simulink model "OpenLoopSys"  (Simulink 8.4)
settings: Solver=ode45  StartTime=0.0  StopTime=60.0  RelTol=1e-3
values from neighbouring files (symbols this model uses):
  g = 9.81    [heli.m]
  Je = 2*m1*(l1^2)+m2*(l3^2)    (= 0.0023885)    [heli.m]
  Jt = Je    (= 0.0023885)    [heli.m]
  l1 = 0.110    (= 0.11)    [heli.m]
  l3 = 0.108    [heli.m]
  m1 = 0.0505    [heli.m]
  m2 = 0.100    (= 0.1)    [heli.m]
settings Model: Creator=bjones  LastModifiedBy=bjones
settings DebuggingCC: SolverPrmCheckMsg=none

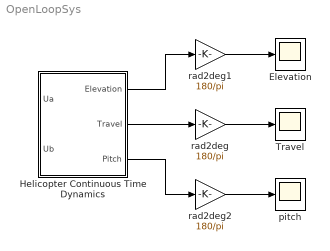
== system OpenLoopSys ==
  Elevation : Scope
      settings: TimeRange=60  YMin=-50  YMax=30  SaveName=elev
  Helicopter Continuous Time Dynamics : Subsystem
  Travel : Scope
      settings: TimeRange=60  YMin=-150  YMax=300  SaveName=trav
  pitch : Scope
      settings: TimeRange=60  YMin=-25  YMax=20  SaveName=pitch
  rad2deg : Gain  Gain=180/pi  SaturateOnIntegerOverflow=on  OutDataTypeStr=Inherit: Same as input  ParamDataTypeStr=Inherit: Same as input
  rad2deg1 : Gain  Gain=180/pi  SaturateOnIntegerOverflow=on  OutDataTypeStr=Inherit: Same as input  ParamDataTypeStr=Inherit: Same as input
  rad2deg2 : Gain  Gain=180/pi  SaturateOnIntegerOverflow=on  OutDataTypeStr=Inherit: Same as input  ParamDataTypeStr=Inherit: Same as input
  wires:
  rad2deg/1 -> Travel/1
  rad2deg1/1 -> Elevation/1
  Helicopter Continuous Time Dynamics/2(Travel) -> rad2deg/1
  Helicopter Continuous Time Dynamics/1(Elevation) -> rad2deg1/1
  rad2deg2/1 -> pitch/1
  Helicopter Continuous Time Dynamics/3(Pitch) -> rad2deg2/1

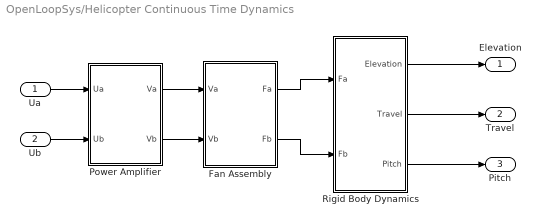
== system OpenLoopSys/Helicopter Continuous Time Dynamics ==
  Ua : Inport
  Ub : Inport  Port=2
  Fan Assembly : Subsystem
  Power Amplifier : Subsystem
  Rigid Body Dynamics : Subsystem
  Elevation : Outport
  Travel : Outport  Port=2
  Pitch : Outport  Port=3
  wires:
  Power Amplifier/1(Va) -> Fan Assembly/1(Va)
  Power Amplifier/2(Vb) -> Fan Assembly/2(Vb)
  Rigid Body Dynamics/1(Elevation) -> Elevation/1
  Rigid Body Dynamics/3(Pitch) -> Pitch/1
  Fan Assembly/2(Fb) -> Rigid Body Dynamics/2(Fb)
  Ua/1 -> Power Amplifier/1(Ua)
  Ub/1 -> Power Amplifier/2(Ub)
  Rigid Body Dynamics/2(Travel) -> Travel/1
  Fan Assembly/1(Fa) -> Rigid Body Dynamics/1(Fa)

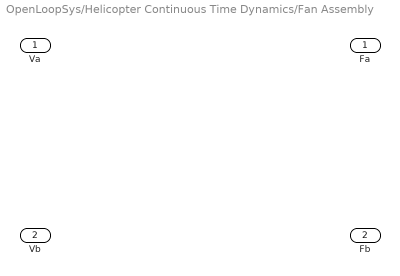
== system OpenLoopSys/Helicopter Continuous Time Dynamics/Fan Assembly ==
  Va : Inport
  Vb : Inport  Port=2
  Fa : Outport
  Fb : Outport  Port=2

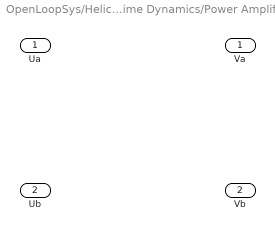
== system OpenLoopSys/Helicopter Continuous Time Dynamics/Power Amplifier ==
  Ua : Inport
  Ub : Inport  Port=2
  Va : Outport
  Vb : Outport  Port=2

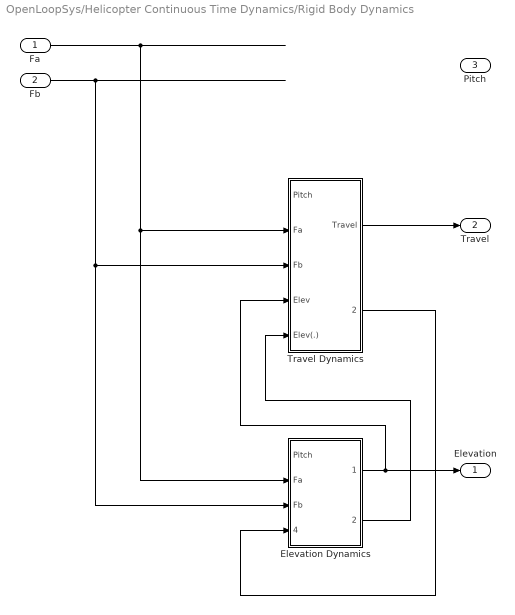
== system OpenLoopSys/Helicopter Continuous Time Dynamics/Rigid Body Dynamics ==
  Fa : Inport
  Fb : Inport  Port=2
  Elevation Dynamics : Subsystem
  Travel Dynamics : Subsystem
  Elevation : Outport
  Travel : Outport  Port=2
  Pitch : Outport  Port=3
  wires:
  Fa/1 -> Travel Dynamics/2(Fa), Elevation Dynamics/2(Fa)
  Fb/1 -> Elevation Dynamics/3(Fb), Travel Dynamics/3(Fb)
  Travel Dynamics/1(Travel) -> Travel/1
  Elevation Dynamics/1(Elevation) -> Elevation/1, Travel Dynamics/4(Elev)
  ? -> Travel Dynamics/1(Pitch), Elevation Dynamics/1(Pitch), Pitch/1
  Travel Dynamics/2(Travel(.)) -> Elevation Dynamics/4(Travel(.))
  Elevation Dynamics/2(Elevation(.)) -> Travel Dynamics/5(Elev(.))

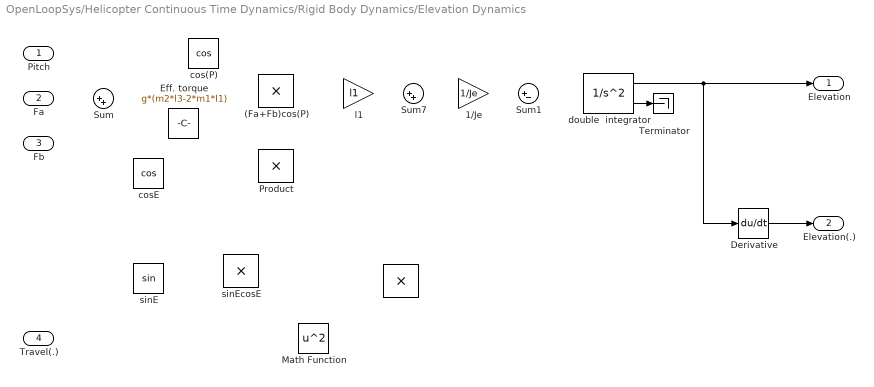
== system OpenLoopSys/Helicopter Continuous Time Dynamics/Rigid Body Dynamics/Elevation Dynamics ==
  Pitch : Inport
  Fa : Inport  Port=2
  Fb : Inport  Port=3
  Travel(.) : Inport  Port=4
  " " : Product  SaturateOnIntegerOverflow=on  RndMeth=Zero  InputSameDT=on  OutDataTypeStr=Inherit: Same as first input
  (Fa+Fb)cos(P) : Product  SaturateOnIntegerOverflow=on  RndMeth=Zero  InputSameDT=on  OutDataTypeStr=Inherit: Same as first input
  1/Je : Gain  Gain=1/Je  SaturateOnIntegerOverflow=on  OutDataTypeStr=Inherit: Same as input  ParamDataTypeStr=Inherit: Same as input
  Derivative : Derivative
  Eff. torque : Constant  Value=g*(m2*l3-2*m1*l1)
  Math Function : Math  Operator=square  SaturateOnIntegerOverflow=on
  Product : Product  SaturateOnIntegerOverflow=on  RndMeth=Zero  InputSameDT=on  OutDataTypeStr=Inherit: Same as first input
  Sum : Sum  Inputs=|++  SaturateOnIntegerOverflow=on  InputSameDT=on  OutDataTypeStr=Inherit: Same as first input
  Sum1 : Sum  Inputs=|+-  SaturateOnIntegerOverflow=on  InputSameDT=on  OutDataTypeStr=Inherit: Same as first input
  Sum7 : Sum  Inputs=|++  SaturateOnIntegerOverflow=on  InputSameDT=on  OutDataTypeStr=Inherit: Same as first input
  Terminator : Terminator
  cos(P) : Trigonometry  Operator=cos
  cosE : Trigonometry  Operator=cos
  double  integrator : SecondOrderIntegrator  ICX=e_lim_l  LimitX=on  UpperLimitX=e_lim_u  LowerLimitX=e_lim_l  LimitDXDT=on  UpperLimitDXDT=2*pi  LowerLimitDXDT=-2*pi
  l1 : Gain  Gain=l1  SaturateOnIntegerOverflow=on  OutDataTypeStr=Inherit: Same as input  ParamDataTypeStr=Inherit: Same as input
  sinE : Trigonometry
  sinEcosE : Product  SaturateOnIntegerOverflow=on  RndMeth=Zero  InputSameDT=on  OutDataTypeStr=Inherit: Same as first input
  Elevation : Outport
  Elevation(.) : Outport  Port=2
  wires:
  double  integrator/1 -> Elevation/1, Derivative/1
  Derivative/1 -> Elevation(.)/1
  double  integrator/2 -> Terminator/1

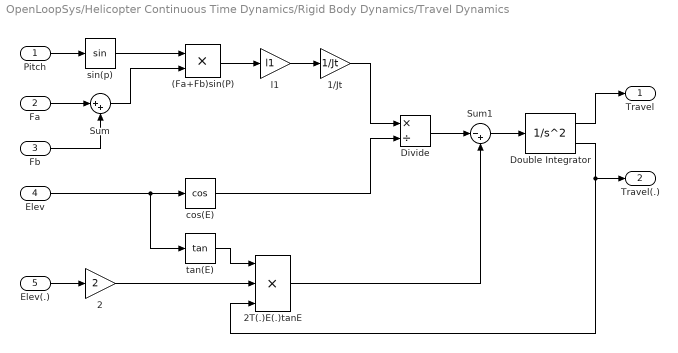
== system OpenLoopSys/Helicopter Continuous Time Dynamics/Rigid Body Dynamics/Travel Dynamics ==
  Pitch : Inport
  Fa : Inport  Port=2
  Fb : Inport  Port=3
  Elev : Inport  Port=4
  Elev(.) : Inport  Port=5
  (Fa+Fb)sin(P) : Product  SaturateOnIntegerOverflow=on  RndMeth=Zero  InputSameDT=on  OutDataTypeStr=Inherit: Same as first input
  1/Jt : Gain  Gain=1/Jt  SaturateOnIntegerOverflow=on  OutDataTypeStr=Inherit: Same as input  ParamDataTypeStr=Inherit: Same as input
  2 : Gain  Gain=2  SaturateOnIntegerOverflow=on  OutDataTypeStr=Inherit: Same as input  ParamDataTypeStr=Inherit: Same as input
  2T(.)E(.)tanE : Product  Inputs=3  SaturateOnIntegerOverflow=on  RndMeth=Zero  InputSameDT=on  OutDataTypeStr=Inherit: Same as first input
  Divide : Product  Inputs=*/
  Double Integrator : SecondOrderIntegrator  UpperLimitX=1  LowerLimitX=0  LimitDXDT=on  UpperLimitDXDT=2  LowerLimitDXDT=-2
  Sum : Sum  Inputs=|++  SaturateOnIntegerOverflow=on  InputSameDT=on  OutDataTypeStr=Inherit: Same as first input
  Sum1 : Sum  Inputs=|-+  SaturateOnIntegerOverflow=on  InputSameDT=on  OutDataTypeStr=Inherit: Same as first input
  cos(E) : Trigonometry  Operator=cos
  l1 : Gain  Gain=l1  SaturateOnIntegerOverflow=on  OutDataTypeStr=Inherit: Same as input  ParamDataTypeStr=Inherit: Same as input
  sin(p) : Trigonometry
  tan(E) : Trigonometry  Operator=tan
  Travel : Outport
  Travel(.) : Outport  Port=2
  wires:
  Double Integrator/1 -> Travel/1
  sin(p)/1 -> (Fa+Fb)sin(P)/1
  (Fa+Fb)sin(P)/1 -> l1/1
  Pitch/1 -> sin(p)/1
  Fa/1 -> Sum/1
  Fb/1 -> Sum/2
  Sum/1 -> (Fa+Fb)sin(P)/2
  l1/1 -> 1/Jt/1
  Elev/1 -> cos(E)/1, tan(E)/1
  1/Jt/1 -> Divide/1
  cos(E)/1 -> Divide/2
  Double Integrator/2 -> Travel(.)/1, 2T(.)E(.)tanE/3
  tan(E)/1 -> 2T(.)E(.)tanE/1
  Elev(.)/1 -> 2/1
  2/1 -> 2T(.)E(.)tanE/2
  Divide/1 -> Sum1/1
  Sum1/1 -> Double Integrator/1
  2T(.)E(.)tanE/1 -> Sum1/2
